simulink model "Linear_Model"  (R2024b)
settings: Solver=VariableStepAuto  StartTime=0.0  StopTime=10.0  RelTol=1e-3
PreLoadFcn:
  | vehicle_var
values from neighbouring files (symbols this model uses):
  A = [ -(Ca_f + Ca_r)/(M*vx),  -(Ca_f*lf - Ca_r*lr)/(M*vx)-vx,  0,  0 ... (first row only)    [vehicle_var.m]
  B = [ ... (first row only)    [vehicle_var.m]
  C = [ ... (first row only)    [vehicle_var.m]
  D = [ 0 ; 0 ]    [vehicle_var.m]
libraries: simulink x2
settings Model: Creator=Antonio  LastModifiedBy=Antonio
settings DataIOCC: InspectSignalLogs=on  LoggingToFile=on

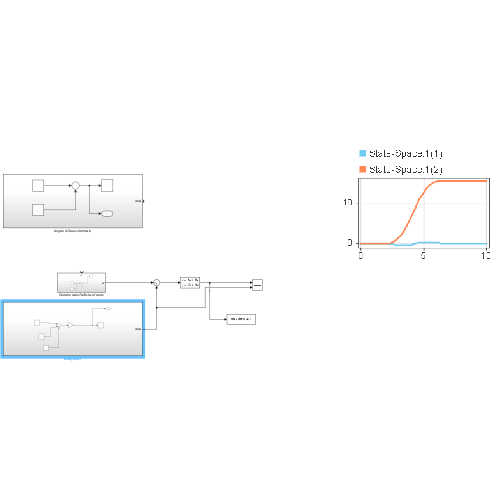
[thumbnail: Simulink's stored preview of the top-level diagram]
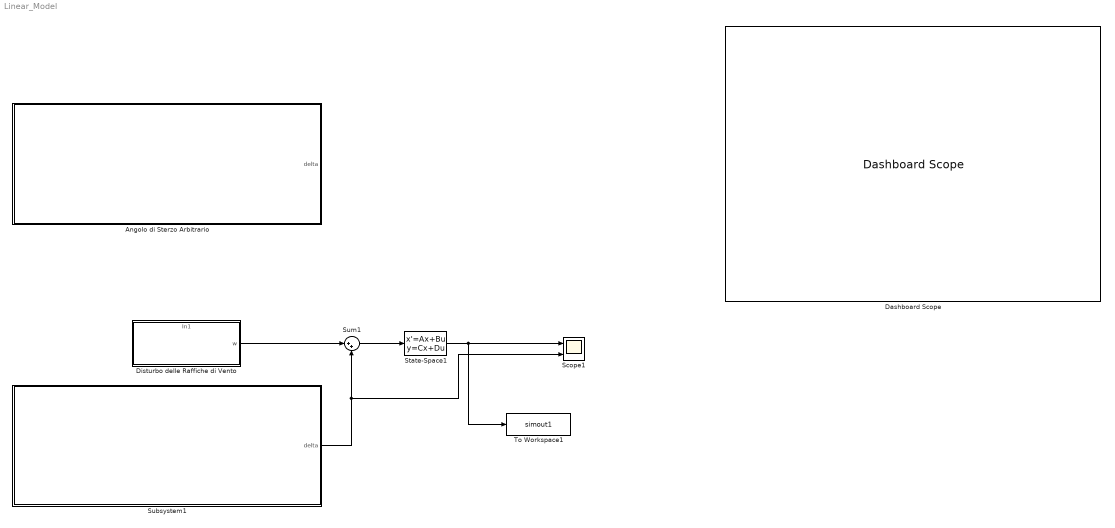
== system Linear_Model ==
  Angolo di Sterzo Arbitrario : Subsystem
  Dashboard Scope : DashboardScope
  Disturbo delle Raffiche di Vento : Subsystem
      settings: PortSchema="{\"entries\":[{\"content\":{\"sides\":[{\"content\":{},\"type\":\"ConnectorPlacement.EquallySpacedRectSide\",\"uuid\":\"bb16746b-4cff-4599-943a-292f777770d9\"},{\"content\":{\"connectorIds\":[\"Out1\"],\"side\":\"RIGHT\"},\"type\":\"ConnectorPlacement.EquallySpacedRectSide\",\"uuid\":\"a29f9bb7-7b51-45c6-8f9a-557f17f85f71\"},{\"content\":{\"connectorIds\":[\"In1\"],\"side\":\"TOP\"},\"type\":\"ConnectorPlacement.EquallySpacedRectSide\",\"uuid\":\"a3ef89ec-9232-4880-b59f-57390fe249bf\"}]},\"type\":\"ConnectorPlacement.EquallySpacedConnector\",\"uuid\":\"b7c3f02b-dabd-429b-b8e6-a94e8be84a22\"}],\"packageUris\":[\"http://schema.mathworks.com/mf0/Connector/R2020b\"],\"version\":\"1.0\"}"
  Scope1 : Scope  NumInputPorts=2
  State-Space1 : StateSpace  A=A  B=B  C=C  D=D  InitialCondition=0
  Subsystem1 : Subsystem
  Sum1 : Sum  Inputs=|++
  To Workspace1 : ToWorkspace  VariableName=simout1  SaveFormat=Timeseries  SampleTime=-1
  wires:
  Subsystem1/1(delta) -> Scope1/2, Sum1/2
  Sum1/1 -> State-Space1/1
  State-Space1/1 -> To Workspace1/1, Scope1/1
  Disturbo delle Raffiche di Vento/1(w) -> Sum1/1

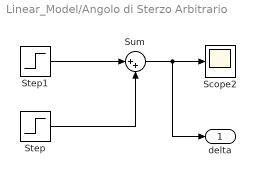
== system Linear_Model/Angolo di Sterzo Arbitrario ==
  Scope2 : Scope
  Step : Step  Time=4  Before=4  After=0  SampleTime=0
  Step1 : Step  Time=2  After=4  SampleTime=0
  Sum : Sum  Inputs=|++
  delta : Outport
  wires:
  Sum/1 -> delta/1, Scope2/1
  Step1/1 -> Sum/1
  Step/1 -> Sum/2

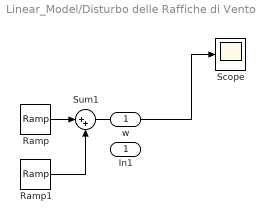
== system Linear_Model/Disturbo delle Raffiche di Vento ==
  In1 : Inport
  Ramp : simulink/Sources/Ramp  slope=-8  start=2  InitialOutput=0
  Ramp1 : simulink/Sources/Ramp  slope=8  start=3  InitialOutput=9
  Scope : Scope
  Sum1 : Sum  Inputs=|++
  w : Outport
  wires:
  Ramp/1 -> Sum1/1
  Sum1/1 -> Scope/1
  Ramp1/1 -> Sum1/2

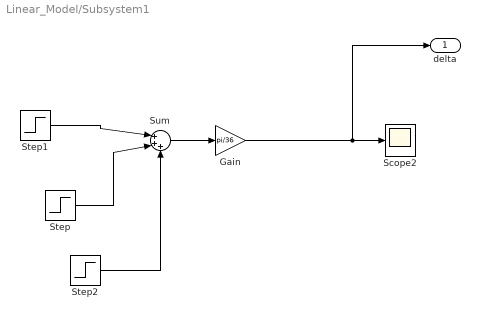
== system Linear_Model/Subsystem1 ==
  Gain : Gain  Gain=pi/36
  Scope2 : Scope
  Step : Step  Time=4  After=-2  SampleTime=0
  Step1 : Step  Time=2  SampleTime=0
  Step2 : Step  Time=6  SampleTime=0
  Sum : Sum  Inputs=|+++
  delta : Outport
  wires:
  Sum/1 -> Gain/1
  Step1/1 -> Sum/1
  Gain/1 -> delta/1, Scope2/1
  Step/1 -> Sum/2
  Step2/1 -> Sum/3
